simulink model "BLDC_PMSM_drive_with_Hall_sensor_6_step_commutation"  (R2024a)
settings: Solver=ode15s  StartTime=0.0  StopTime=5  MaxStep=1e-5  MinStep=1e-6  RelTol=1e-3
libraries: spsDCVoltageSourceLib x1, spsPermanentMagnetSynchronousMachineLib x1, spsUniversalBridgeLib x1, sps_lib x1
settings Model: Creator=haris  LastModifiedBy=haris

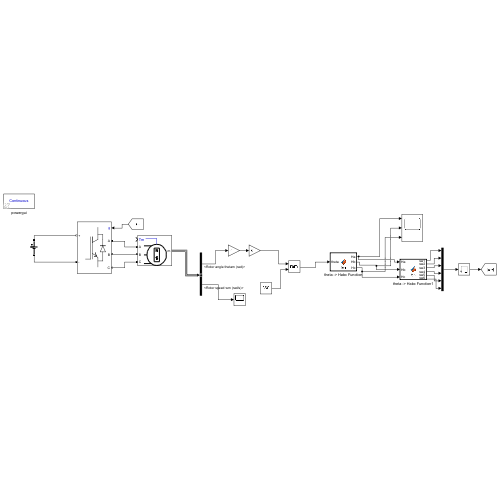
[thumbnail: Simulink's stored preview of the top-level diagram]
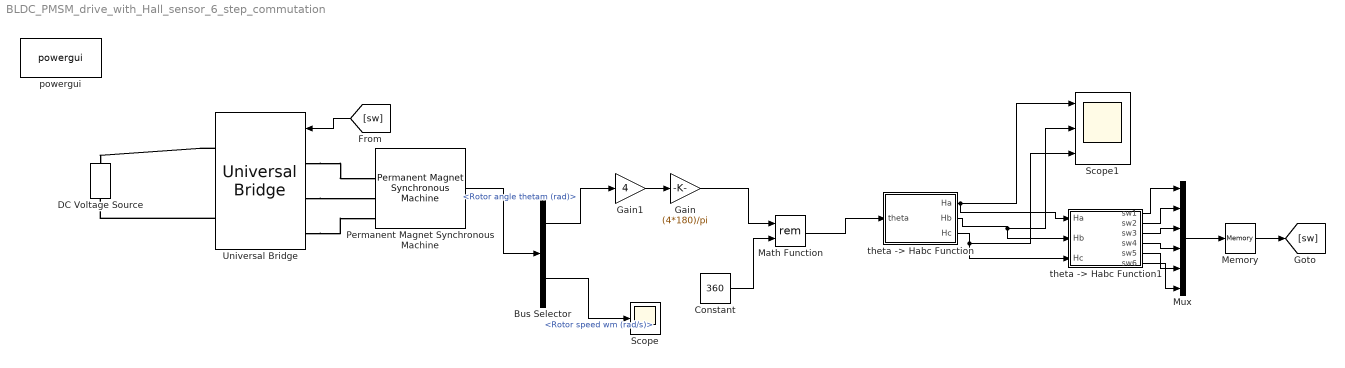
== system BLDC_PMSM_drive_with_Hall_sensor_6_step_commutation ==
  Bus Selector : BusSelector  OutputSignals=Rotor angle thetam (rad),Rotor speed wm (rad/s)
  Constant : Constant  Value=360
  DC Voltage Source : spsDCVoltageSourceLib/DC Voltage Source  Amplitude=100  Measurements=None
  Gain : Gain  Gain=(4*180)/pi
  Gain1 : Gain  Gain=4
  Math Function : Math  Operator=rem
  Memory : Memory
  Mux : Mux  Inputs=6
  Permanent Magnet Synchronous Machine : spsPermanentMagnetSynchronousMachineLib/Permanent Magnet Synchronous Machine  NbPhases=3  FluxDistribution=Trapezoidal  RotorType=Round  MechanicalLoad=Torque Tm  PresetModel=No  ShowDetailedParameters=on  MeasurementBus=off  Resistance=0.0485  Inductance=0.000395  dqInductances=[8.5e-3,8.5e-3]  La=0.000395  MachineConstant=Flux linkage established by magnets (V.s)  Flux=0.1194  VoltageCst=100.0283  TorqueCst=0.9552  Flat=120  Mechanical=[0.0027 0.0004924 4 0]  PolePairs=4  InitialConditions=[0,0, 0,0]  InitialConditions5ph=[0 0 0 0 0 0]  RefAngle=90 degrees behind phase A axis (modified Park)  IterativeDiscreteModel=Trapezoidal non iterative  TsBlock=-1  TsPowergui=0
  Scope : Scope
  Scope1 : Scope  NumInputPorts=3
  Universal Bridge : spsUniversalBridgeLib/Universal Bridge  Arms=3  SnubberResistance=1e-5  SnubberCapacitance=inf  Device=IGBT / Diodes  Ron=1e-3  Lon=0  ForwardVoltages="[  0  0  ]"  ForwardVoltage=0  GTOparameters=[ 10e-6 , 20e-6 ]  IGBTparameters=[ 1e-6 , 2e-6 ]  Measurements=None  Measurements_2=None  converterType=Rectifier
  powergui : sps_lib/powergui  Priority=1  SimulationMode=Continuous  SampleTime=50e-6  frequency=60  Iterations=50  frequencyindice=0  Pbase=100e6  ErrMax=1e-4  UnitsV=kV  UnitsW=MW  buscounter=0  FunctionMessages=off  echomessages=off  EnableUseOfTLC=off  CurrentSourceSwitches=off  DisableSnubberDevices=off  DisableRonSwitches=off  DisableVfSwitches=off  DisplayEquations=off  AutomaticDiscreteSolvers=off  SolverType=Tustin/Backward Euler (TBE)  Interpol=off  ExternalGateDelay=off  methode=off  Ts=100  x0status=blocks  SPID=on  SwTol=0  HookPort=off  NonlinearTolerance=1e-4  nMaxIteration=100  ContinueOnMaxIteration=off  RestoreLinks=warning  ResistiveCurrentMeasurement=off  Frange=[0:2:500]  Ylog=off  Xlog=on  ShowGrid=off  save=off  variable=ZData  structure=0  ZoomFFT=off  StartTime=0.0  cycles=1  DisplayStyle=1  fundamental=60  FreqAxis=off  MaxFrequency=1000  frequencyindicesteady=1  RmsSteady=1  display=off
  "theta -> Habc Function" : MATLAB Function  TreatAsAtomicUnit=on
  "theta -> Habc Function1" : MATLAB Function  TreatAsAtomicUnit=on
  wires:
  Permanent Magnet Synchronous Machine/1 -> Bus Selector/1
  Bus Selector/2 -> Scope/1  "<Rotor speed wm (rad/s)>"
  Constant/1 -> Math Function/2
  "theta -> Habc Function1"/1(sw1) -> Mux/1
  "theta -> Habc Function1"/2(sw2) -> Mux/2
  "theta -> Habc Function1"/3(sw3) -> Mux/3
  "theta -> Habc Function1"/4(sw4) -> Mux/4
  "theta -> Habc Function1"/5(sw5) -> Mux/5
  "theta -> Habc Function1"/6(sw6) -> Mux/6
  "theta -> Habc Function"/1(Ha) -> "theta -> Habc Function1"/1(Ha), Scope1/1
  "theta -> Habc Function"/2(Hb) -> Scope1/2, "theta -> Habc Function1"/2(Hb)
  "theta -> Habc Function"/3(Hc) -> Scope1/3, "theta -> Habc Function1"/3(Hc)
  [sw] -> Universal Bridge/1
  Mux/1 -> Memory/1
  Memory/1 -> [sw]
  Bus Selector/1 -> Gain1/1  "<Rotor angle thetam (rad)>"
  Gain1/1 -> Gain/1
  Gain/1 -> Math Function/1
  Math Function/1 -> "theta -> Habc Function"/1(theta)
  connections:
  Universal Bridge/RConn1 -- DC Voltage Source/RConn1
  Universal Bridge/RConn2 -- DC Voltage Source/LConn1
  Universal Bridge/LConn2 -- Permanent Magnet Synchronous Machine/LConn2
  Universal Bridge/LConn1 -- Permanent Magnet Synchronous Machine/LConn1
  Universal Bridge/LConn3 -- Permanent Magnet Synchronous Machine/LConn3

== matlab function BLDC_PMSM_drive_with_Hall_sensor_6_step_commutation/theta -> Habc Function1 ==
  data: Ha input; sw1 output; Hb input; Hc input; sw2 output; sw3 output; sw4 output; sw5 output; sw6 output
function [sw1, sw2, sw3, sw4, sw5, sw6] = fcn(Ha, Hb, Hc)
    % CORRECTED BLDC 6-Step Commutation Logic
    % Universal Bridge connections:
    % sw1 = A+ (top), sw2 = A- (bottom)
    % sw3 = B+ (top), sw4 = B- (bottom)  
    % sw5 = C+ (top), sw6 = C- (bottom)
    
    % Initialize all switches to 0 (OFF)
    sw1=0; sw2=0; sw3=0; sw4=0; sw5=0; sw6=0;
    
    % 6-Step Commutation Sequence
    if Ha==1 && Hb==0 && Hc==1      % Sector 1 (0-60°)
        sw1=1; sw6=1;               % A+ and C-
        
    elseif Ha==1 && Hb==0 && Hc==0  % Sector 2 (60-120°)
        sw1=1; sw4=1;               % A+ and B- (FIXED)
        
    elseif Ha==1 && Hb==1 && Hc==0  % Sector 3 (120-180°)
        sw3=1; sw6=1;               % B+ and C- (FIXED)
        
    elseif Ha==0 && Hb==1 && Hc==0  % Sector 4 (180-240°)
        sw3=1; sw2=1;               % B+ and A- (FIXED)
        
    elseif Ha==0 && Hb==1 && Hc==1  % Sector 5 (240-300°)
        sw5=1; sw2=1;               % C+ and A- (FIXED)
        
    elseif Ha==0 && Hb==0 && Hc==1  % Sector 6 (300-360°)
        sw5=1; sw4=1;               % C+ and B- (FIXED)
    end
end

== matlab function BLDC_PMSM_drive_with_Hall_sensor_6_step_commutation/theta -> Habc Function ==
  data: theta input; Ha output; Hb output; Hc output
function [Ha, Hb, Hc] = fcn(theta)
    % Translates 0-360 electrical degrees into 120-degree Hall signals

    if theta >= 0 && theta < 60
        Ha=1; Hb=0; Hc=1;
    elseif theta >= 60 && theta < 120
        Ha=1; Hb=0; Hc=0;
    elseif theta >= 120 && theta < 180
        Ha=1; Hb=1; Hc=0;
    elseif theta >= 180 && theta < 240
        Ha=0; Hb=1; Hc=0;
    elseif theta >= 240 && theta < 300
        Ha=0; Hb=1; Hc=1;
    elseif theta >= 300 && theta <= 360
        Ha=0; Hb=0; Hc=1;
    else
        % Default/Error state - all sensors off
        Ha=0; Hb=0; Hc=0;
    end
end
